simulink model "SITRA_Simscape_Hardware"  (R2026a)
settings: Solver=ode15s  StartTime=0  StopTime=600  MaxStep=1.0
InitFcn:
  | init_simscape_workspace;
libraries: fl_lib x1, nesl_utility x1
settings Model: Creator=saisi  LastModifiedBy=saisi

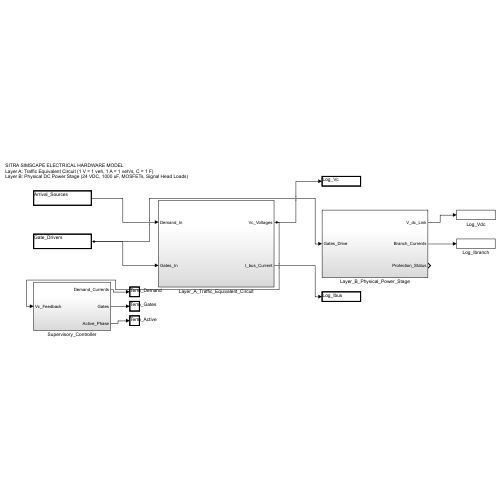
[thumbnail: Simulink's stored preview of the top-level diagram]
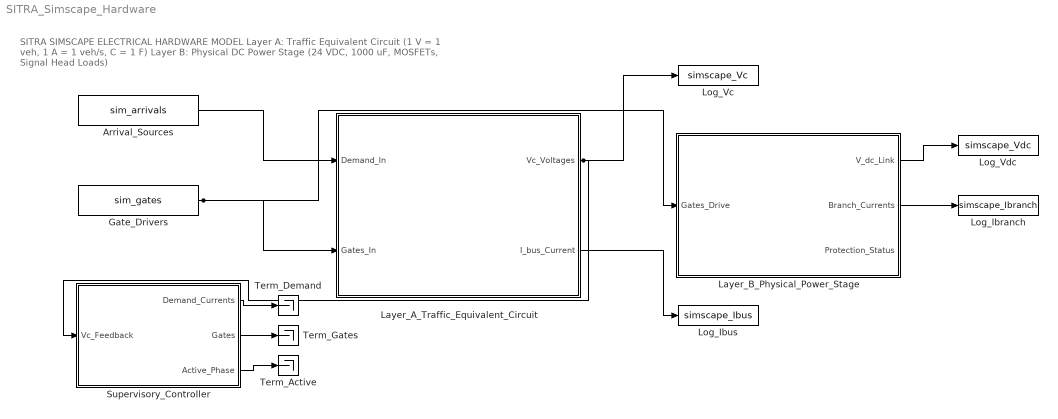
== system SITRA_Simscape_Hardware ==
  note: SITRA SIMSCAPE ELECTRICAL HARDWARE MODEL
      | Layer A: Traffic Equivalent Circuit (1 V = 1 veh, 1 A = 1 veh/s, C = 1 F)
      | Layer B: Physical DC Power Stage (24 VDC, 1000 uF, MOSFETs, Signal Head Loads)
  Arrival_Sources : FromWorkspace  VariableName=sim_arrivals  SampleTime=1  Interpolate=off  OutputAfterFinalValue=Holding final value
  Gate_Drivers : FromWorkspace  VariableName=sim_gates  SampleTime=1  Interpolate=off  OutputAfterFinalValue=Holding final value
  Layer_A_Traffic_Equivalent_Circuit : Subsystem
  Layer_B_Physical_Power_Stage : Subsystem
  Log_Ibranch : ToWorkspace  VariableName=simscape_Ibranch  SampleTime=1
  Log_Ibus : ToWorkspace  VariableName=simscape_Ibus  SampleTime=1
  Log_Vc : ToWorkspace  VariableName=simscape_Vc  SampleTime=1
  Log_Vdc : ToWorkspace  VariableName=simscape_Vdc  SampleTime=1
  Supervisory_Controller : Subsystem
  Term_Active : Terminator
  Term_Demand : Terminator
  Term_Gates : Terminator
  wires:
  Arrival_Sources/1 -> Layer_A_Traffic_Equivalent_Circuit/1(Demand_In)
  Gate_Drivers/1 -> Layer_A_Traffic_Equivalent_Circuit/2(Gates_In), Layer_B_Physical_Power_Stage/1(Gates_Drive)
  Layer_A_Traffic_Equivalent_Circuit/1(Vc_Voltages) -> Supervisory_Controller/1(Vc_Feedback), Log_Vc/1
  Supervisory_Controller/1(Demand_Currents) -> Term_Demand/1
  Supervisory_Controller/2(Gates) -> Term_Gates/1
  Supervisory_Controller/3(Active_Phase) -> Term_Active/1
  Layer_A_Traffic_Equivalent_Circuit/2(I_bus_Current) -> Log_Ibus/1
  Layer_B_Physical_Power_Stage/1(V_dc_Link) -> Log_Vdc/1
  Layer_B_Physical_Power_Stage/2(Branch_Currents) -> Log_Ibranch/1

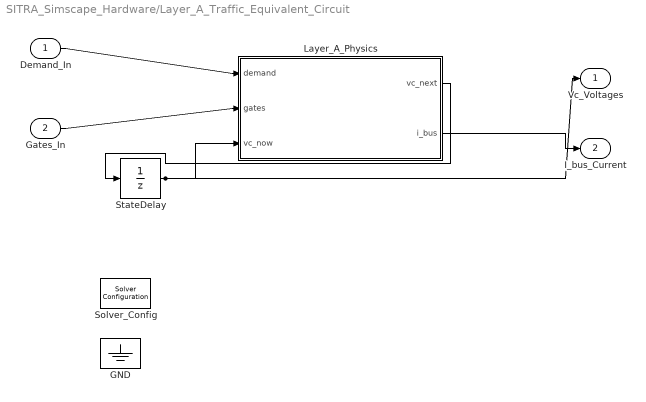
== system SITRA_Simscape_Hardware/Layer_A_Traffic_Equivalent_Circuit ==
  Demand_In : Inport
  Gates_In : Inport  Port=2
  GND : fl_lib/Electrical/Electrical Elements/Electrical Reference
  Layer_A_Physics : MATLAB Function  TreatAsAtomicUnit=on
  Solver_Config : nesl_utility/Solver Configuration  PhysicalDomain=network_engine_domain  SubClassName=solver  LeftPortType=input  RightPortType=generic  Tones=[]  Harmonics=[]  SimulateNoise=off  Profile=off  UseLocalSampling=off  EnableSwitchedLinearOptims=on  FrequencyDomain=off  UseCCode=off  RelTol=0.001  AbsTol=0.001  MinStep=1e-09  ToWorkspace=off  RevertToSquareIcSolve=off  NumHomotopyIterations=100  PhasorMode=off  PhasorModeNumHarmonics=1  ConsistencySolver=NEWTON_XTOL_AFTER_FTOL  CanonicalOrdering=CANONICAL  OptimizeIntermediates=OPTIMIZED  IndexReductionMethod=DerivativeReplacement  DoDC=off  ResidualTolerance=1e-09  ConsistencyTolSource=GLOBAL  ConsistencyAbsTol=0.001  ConsistencyRelTol=0.001  ConsistencyTolFactor=0.001  UseLocalSolver=off  LocalSolverChoice=NE_BACKWARD_EULER_ADVANCER  ResolveIndetEquations=on  FunctionEvalNumThread=1  LocalSolverSampleTime=0.001  DoFixedCost=off  MaxNonlinIter=3  MaxModeIter=2  ComputeImpulses=off  ImpulseIterations=2  LinearAlgebra=auto  LinearAlgebraNumThread=0  EquationFormulation=NE_TIME_EF  DelaysMemoryBudget=1024  AutomaticFiltering=on  FilteringTimeConstant=0.001  PartitionStorageMethod=AS_NEEDED  PartitionMemoryBudget=1024  PartitionMethod=ROBUST  MultibodyUseLocalSolver=off  MultibodyLocalSolverChoice=ODE1  MultibodyLocalSolverSampleTime=0.001
  StateDelay : UnitDelay  InitialCondition=zeros(1,4)
  Vc_Voltages : Outport
  I_bus_Current : Outport  Port=2
  wires:
  Demand_In/1 -> Layer_A_Physics/1(demand)
  Gates_In/1 -> Layer_A_Physics/2(gates)
  StateDelay/1 -> Layer_A_Physics/3(vc_now), Vc_Voltages/1
  Layer_A_Physics/1(vc_next) -> StateDelay/1
  Layer_A_Physics/2(i_bus) -> I_bus_Current/1

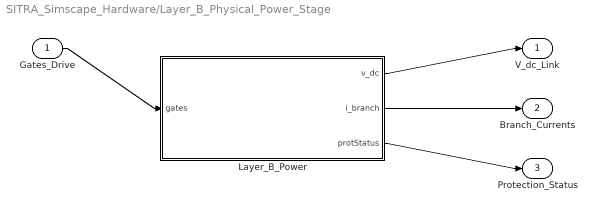
== system SITRA_Simscape_Hardware/Layer_B_Physical_Power_Stage ==
  Gates_Drive : Inport
  Layer_B_Power : MATLAB Function  TreatAsAtomicUnit=on
  V_dc_Link : Outport
  Branch_Currents : Outport  Port=2
  Protection_Status : Outport  Port=3
  wires:
  Gates_Drive/1 -> Layer_B_Power/1(gates)
  Layer_B_Power/1(v_dc) -> V_dc_Link/1
  Layer_B_Power/2(i_branch) -> Branch_Currents/1
  Layer_B_Power/3(protStatus) -> Protection_Status/1

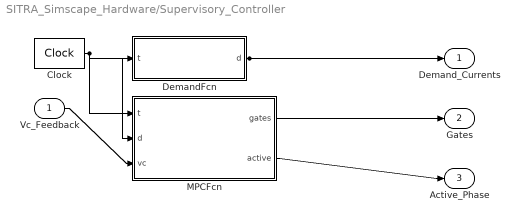
== system SITRA_Simscape_Hardware/Supervisory_Controller ==
  Vc_Feedback : Inport
  Clock : DigitalClock
  DemandFcn : MATLAB Function  TreatAsAtomicUnit=on
  MPCFcn : MATLAB Function  TreatAsAtomicUnit=on
  Demand_Currents : Outport
  Gates : Outport  Port=2
  Active_Phase : Outport  Port=3
  wires:
  Clock/1 -> DemandFcn/1(t), MPCFcn/1(t)
  DemandFcn/1(d) -> Demand_Currents/1, MPCFcn/2(d)
  Vc_Feedback/1 -> MPCFcn/3(vc)
  MPCFcn/1(gates) -> Gates/1
  MPCFcn/2(active) -> Active_Phase/1

== matlab function SITRA_Simscape_Hardware/Supervisory_Controller/MPCFcn ==
  data: t input; gates output; d input; vc input; active output
function [gates, active] = mpcController(t, d, vc)
n = 3;
feedingBranches = [1 2 3];
yellow = 3;
cycleLength = 63;
minGreen = 12;
maxGreen = 30;
totalGreen = cycleLength - n*yellow;
base = minGreen * ones(1, n);
remaining = totalGreen - sum(base);
q3 = max(vc(1:n), 0);
demand = max(reshape(d, 1, 3), 0);
score = q3 + 10 * demand;
score(2:3) = score(2:3) + 0.25;
greenTimes = base;
for s = 1:round(remaining)
    room = maxGreen - greenTimes;
    [m, idx] = max(score .* (room > 1e-12));
    if m <= 0, break; end
    greenTimes(idx) = greenTimes(idx) + 1;
    score(idx) = score(idx) * 0.985 + 1e-12;
end
diffGreen = totalGreen - sum(greenTimes);
while abs(diffGreen) > 1e-12
    if diffGreen > 0
        room = maxGreen - greenTimes;
        [mx, idx] = max(room);
        if mx <= 0, break; end
        add = min(diffGreen, mx);
        greenTimes(idx) = greenTimes(idx) + add;
        diffGreen = totalGreen - sum(greenTimes);
    else
        room = greenTimes - minGreen;
        [mx, idx] = max(room);
        if mx <= 0, break; end
        sub = min(-diffGreen, mx);
        greenTimes(idx) = greenTimes(idx) - sub;
        diffGreen = totalGreen - sum(greenTimes);
    end
end
tau = mod(t, cycleLength);
current = 0;
active = 0;
for p = 1:n
    b = p;
    gEnd = current + greenTimes(b);
    yEnd = gEnd + yellow;
    if tau >= current && tau < gEnd
        active = feedingBranches(b);
        break;
    elseif tau >= gEnd && tau < yEnd
        active = 0;
        break;
    end
    current = yEnd;
end
gates = zeros(1, 3);
if active >= 1 && active <= 3
    gates(active) = 1.0;
end
end

== matlab function SITRA_Simscape_Hardware/Supervisory_Controller/DemandFcn ==
  data: t input; d output
function d = demandProfile(t)
normalD = [0.10 0.07 0.05];
surgeD  = [0.30 0.07 0.05];
if t >= 200 && t < 400
    d = surgeD;
else
    d = normalD;
end
end

== matlab function SITRA_Simscape_Hardware/Layer_A_Traffic_Equivalent_Circuit/Layer_A_Physics ==
  data: demand input; vc_next output; gates input; vc_now input; i_bus output
function [vc_next, i_bus] = layerACore(demand, gates, vc_now)
C = [1.0 1.0 1.0 1.0];
cap = [0.65 0.35 0.25 0.45];
dt = 1.0;
vc = reshape(vc_now, 1, 4);
d = reshape(demand, 1, 3);
g = reshape(gates, 1, 3);
i_arr = [d, 0.0];
i_dep = zeros(1, 4);
for b = 1:3
    if g(b) > 0.5
        i_dep(b) = min(cap(b), vc(b) / dt);
    end
end
i_bus = sum(i_dep(1:3));
i_arr(4) = i_bus;
i_dep(4) = min(cap(4), vc(4) / dt);
vc_next = max(zeros(1, 4), vc + (dt ./ C) .* (i_arr - i_dep));
end

== matlab function SITRA_Simscape_Hardware/Layer_B_Physical_Power_Stage/Layer_B_Power ==
  data: gates input; v_dc output; i_branch output; protStatus output
function [v_dc, i_branch, protStatus] = layerBPhysics(gates)
V_source = 24.0; R_s = 0.05;
C_dc = 1000e-6; R_load = 24.0; R_on = 0.025; dt = 1.0;
g = reshape(gates, 1, 3);
act = find(g > 0.5, 1);
if ~isempty(act)
    R_leg = R_load + R_on;
    G_eq = (1 / R_s) + (1 / R_leg);
    V_eq = (V_source / R_s) / G_eq;
    v_dc = V_eq;
    i_branch = zeros(1, 3);
    i_branch(act) = v_dc / R_leg;
else
    v_dc = V_source;
    i_branch = zeros(1, 3);
end
overcurrent = any(i_branch > 2.0);
undervoltage = (v_dc < 18.0);
protStatus = double(overcurrent || undervoltage);
end
